simulink model "prensa_fluidtek"  (R2026b)
settings: Solver=ode15s  StopTime=P.t_fin  MaxStep=1e-4  RelTol=1e-5
InitFcn:
  | if ~exist('P','var'), P = params_prensa(); end
  | if ~exist('cmd','var'), cmd = [0 0; 1 0; 1 1; 4 1; 4 -1; 7 -1; 7 0; 100 0]; end
values from neighbouring files (symbols this model uses):
  P = struct()    [params_prensa.m]
settings Model: Creator=joela  LastModifiedBy=joela

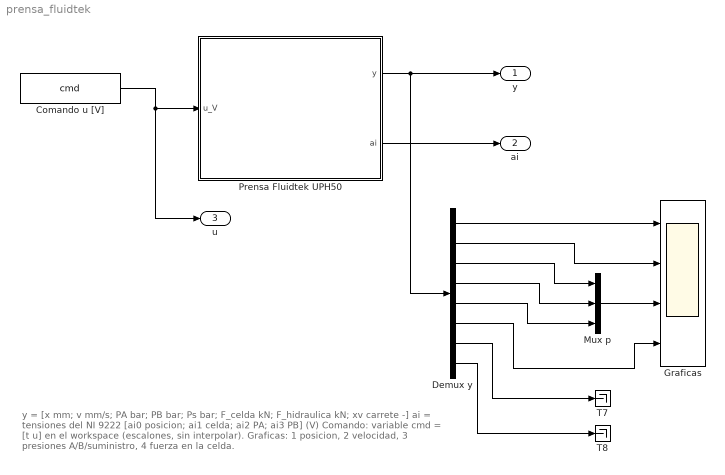
== system prensa_fluidtek ==
  note: y = [x mm; v mm/s; PA bar; PB bar; Ps bar; F_celda kN; F_hidraulica kN; xv carrete -]
      | ai = tensiones del NI 9222 [ai0 posicion; ai1 celda; ai2 PA; ai3 PB] (V)
      | Comando: variable cmd = [t u] en el workspace (escalones, sin interpolar).
      | Graficas: 1 posicion, 2 velocidad, 3 presiones A/B/suministro, 4 fuerza en la celda.
  Comando u [V] : FromWorkspace  VariableName=cmd  Interpolate=off  OutputAfterFinalValue=Holding final value
  Demux y : Demux  Outputs=8
  Graficas : Scope  NumInputPorts=4
  Mux p : Mux  Inputs=3
  Prensa Fluidtek UPH50 : Subsystem
  T7 : Terminator
  T8 : Terminator
  y : Outport
  ai : Outport  Port=2
  u : Outport  Port=3
  wires:
  Comando u [V]/1 -> Prensa Fluidtek UPH50/1(u_V), u/1
  Prensa Fluidtek UPH50/1(y) -> y/1, Demux y/1
  Prensa Fluidtek UPH50/2(ai) -> ai/1
  Demux y/1 -> Graficas/1
  Demux y/2 -> Graficas/2
  Demux y/3 -> Mux p/1
  Demux y/4 -> Mux p/2
  Demux y/5 -> Mux p/3
  Mux p/1 -> Graficas/3
  Demux y/6 -> Graficas/4
  Demux y/7 -> T7/1
  Demux y/8 -> T8/1

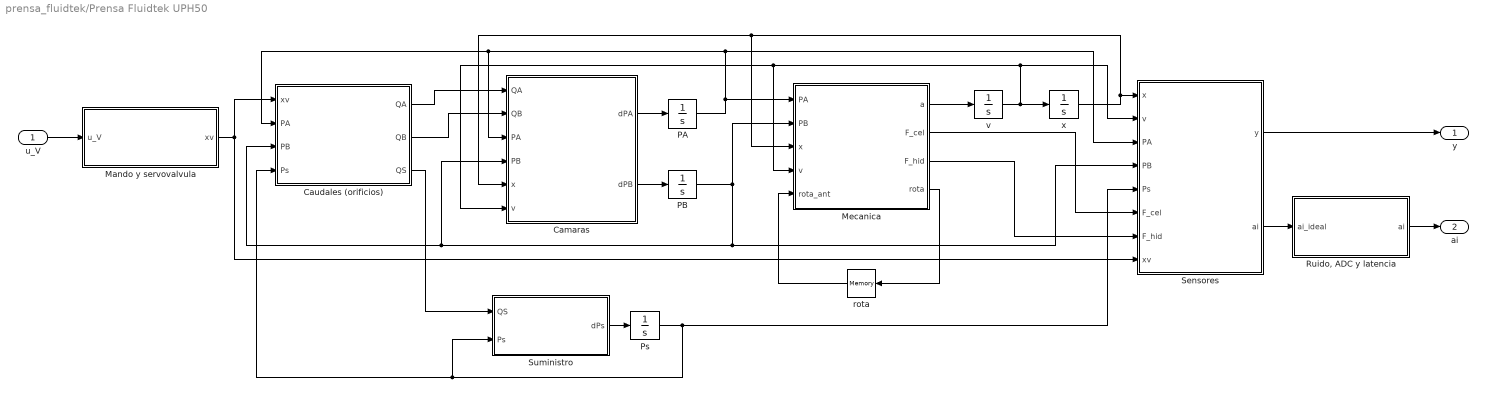
== system prensa_fluidtek/Prensa Fluidtek UPH50 ==
  u_V : Inport
  Camaras : MATLAB Function  TreatAsAtomicUnit=on
  Caudales (orificios) : MATLAB Function  TreatAsAtomicUnit=on
  Mando y servovalvula : Subsystem
  Mecanica : MATLAB Function  TreatAsAtomicUnit=on
  PA : Integrator  InitialCondition=P.PA_ini  LimitOutput=on  UpperSaturationLimit=500e5  LowerSaturationLimit=0
  PB : Integrator  InitialCondition=P.PB_ini  LimitOutput=on  UpperSaturationLimit=500e5  LowerSaturationLimit=0
  Ps : Integrator  InitialCondition=P.Ps_ini  LimitOutput=on  UpperSaturationLimit=400e5  LowerSaturationLimit=0
  "Ruido, ADC y latencia" : Subsystem
  Sensores : MATLAB Function  TreatAsAtomicUnit=on
  Suministro : MATLAB Function  TreatAsAtomicUnit=on
  rota : Memory
  v : Integrator  AbsoluteTolerance=1e-9
  x : Integrator  InitialCondition=P.x_ini  AbsoluteTolerance=1e-10
  y : Outport
  ai : Outport  Port=2
  wires:
  u_V/1 -> Mando y servovalvula/1(u_V)
  Mando y servovalvula/1(xv) -> Caudales (orificios)/1(xv), Sensores/8(xv)
  PA/1 -> Mecanica/1(PA), Camaras/3(PA), Caudales (orificios)/2(PA), Sensores/3(PA)
  PB/1 -> Sensores/4(PB), Camaras/4(PB), Caudales (orificios)/3(PB), Mecanica/2(PB)
  Ps/1 -> Caudales (orificios)/4(Ps), Suministro/2(Ps), Sensores/5(Ps)
  Caudales (orificios)/3(QS) -> Suministro/1(QS)
  Suministro/1(dPs) -> Ps/1
  Caudales (orificios)/1(QA) -> Camaras/1(QA)
  Caudales (orificios)/2(QB) -> Camaras/2(QB)
  x/1 -> Mecanica/3(x), Camaras/5(x), Sensores/1(x)
  v/1 -> x/1, Mecanica/4(v), Camaras/6(v), Sensores/2(v)
  Camaras/1(dPA) -> PA/1
  Camaras/2(dPB) -> PB/1
  rota/1 -> Mecanica/5(rota_ant)
  Mecanica/1(a) -> v/1
  Mecanica/4(rota) -> rota/1
  Mecanica/2(F_cel) -> Sensores/6(F_cel)
  Mecanica/3(F_hid) -> Sensores/7(F_hid)
  Sensores/1(y) -> y/1
  Sensores/2(ai) -> "Ruido, ADC y latencia"/1(ai_ideal)
  "Ruido, ADC y latencia"/1(ai) -> ai/1

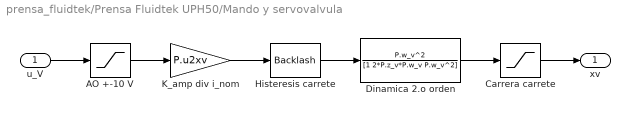
== system prensa_fluidtek/Prensa Fluidtek UPH50/Mando y servovalvula ==
  u_V : Inport
  AO +-10 V : Saturate  UpperLimit=P.u_max  LowerLimit=-P.u_max
  Carrera carrete : Saturate  UpperLimit=1  LowerLimit=-1
  Dinamica 2.o orden : TransferFcn  Numerator=P.w_v^2  Denominator=[1 2*P.z_v*P.w_v P.w_v^2]
  Histeresis carrete : Backlash  BacklashWidth=max(P.histeresis,1e-9)
  K_amp div i_nom : Gain  Gain=P.u2xv
  xv : Outport
  wires:
  u_V/1 -> AO +-10 V/1
  AO +-10 V/1 -> K_amp div i_nom/1
  K_amp div i_nom/1 -> Histeresis carrete/1
  Histeresis carrete/1 -> Dinamica 2.o orden/1
  Dinamica 2.o orden/1 -> Carrera carrete/1
  Carrera carrete/1 -> xv/1

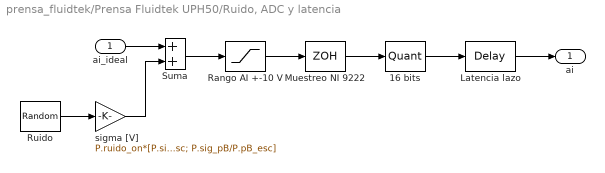
== system prensa_fluidtek/Prensa Fluidtek UPH50/Ruido, ADC y latencia ==
  ai_ideal : Inport
  16 bits : Quantizer  QuantizationInterval=20/2^16
  Latencia lazo : TransportDelay  DelayTime=P.latencia
  Muestreo NI 9222 : ZeroOrderHold  SampleTime=P.Ts_daq
  Rango AI +-10 V : Saturate  UpperLimit=10  LowerLimit=-10
  Ruido : RandomNumber  Seed=[11 12 13 14]  SampleTime=P.Ts_daq
  Suma : Sum
  sigma [V] : Gain  Gain=P.ruido_on*[P.sig_x/P.Kx_sens; P.sig_F/P.KF_sens; P.sig_pA/P.pA_esc; P.sig_pB/P.pB_esc]
  ai : Outport
  wires:
  ai_ideal/1 -> Suma/1
  Ruido/1 -> sigma [V]/1
  sigma [V]/1 -> Suma/2
  Suma/1 -> Rango AI +-10 V/1
  Rango AI +-10 V/1 -> Muestreo NI 9222/1
  Muestreo NI 9222/1 -> 16 bits/1
  16 bits/1 -> Latencia lazo/1
  Latencia lazo/1 -> ai/1

== matlab function prensa_fluidtek/Prensa Fluidtek UPH50/Suministro ==
  data: QS input; dPs output; Ps input; P parameter
function dPs = f_suministro(QS, Ps, P)
%#codegen
% Fuente de presion (Jelali 4.2.4): bomba de caudal constante Qp, limitadora
% tarada en Ps0, capacidad de la manguera P y del acumulador de vejiga.
if P.supply_dyn < 0.5
    dPs = 0;   % presion de suministro ideal y constante
    return
end
Qrv = P.K_rv*max(Ps - P.Ps0, 0);          % limitadora
C = P.V_s/E_lee(Ps, P);                    % aceite en manguera y manifold
if Ps > P.p_acc0                           % acumulador (gas politropico)
    Vg = P.V_acc*(P.p_acc0/Ps)^(1/P.n_acc);
    C = C + Vg/(P.n_acc*Ps);
end
dPs = (P.Qp - QS - Qrv)/C;
end

function E = E_lee(p, P)
% Modulo de compresibilidad efectivo de Lee (Jelali 3.21)
E = P.a1*P.E_max*log10(P.a2*max(p, 1e4)/P.p_max + P.a3);
end

== matlab function prensa_fluidtek/Prensa Fluidtek UPH50/Caudales (orificios) ==
  data: xv input; QA output; PA input; PB input; Ps input; QB output; QS output; P parameter
function [QA, QB, QS] = f_caudales(xv, PA, PB, Ps, P)
%#codegen
% Servovalvula de 4 vias, Jelali & Kroll (2003) ec. 4.5-4.6 (underlap).
% xv: posicion normalizada del carrete [-1,1]; presiones en Pa.
% QA = caudal que ENTRA en la camara A; QB = caudal que ENTRA en la camara B;
% QS = caudal que sale de la fuente de presion.
xe = xv + P.x0;                 % offset de null
a1 = max(P.xu + xe, 0);         % aristas P->A y B->T
a2 = max(P.xu - xe, 0);         % aristas P->B y A->T
QPA = P.Cv*a1*rq(Ps - PA, P.p_lam);
QAT = P.Cv*a2*rq(PA - P.PT, P.p_lam);
QPB = P.Cv*a2*rq(Ps - PB, P.p_lam);
QBT = P.Cv*a1*rq(PB - P.PT, P.p_lam);
QA = QPA - QAT;
QB = QPB - QBT;
QS = QPA + QPB;
end

function q = rq(dp, pl)
% raiz con signo: turbulenta si |dp| >> pl, laminar cerca de cero
q = dp/sqrt(abs(dp) + pl);
end

== matlab function prensa_fluidtek/Prensa Fluidtek UPH50/Camaras ==
  data: QA input; dPA output; QB input; PA input; PB input; x input; v input; dPB output; P parameter
function [dPA, dPB] = f_camaras(QA, QB, PA, PB, x, v, P)
%#codegen
% Dinamica de presion en las camaras, Jelali (2003) ec. 4.51-4.52.
% Volumenes variables con la carrera (4.46-4.47); x=0 vastago retraido.
VA = max(P.VA0 + P.A_A*x, 1e-6);
VB = max(P.VB0 + P.A_B*(P.L_fis - x), 1e-6);
QLi = P.C_Li*(PA - PB);                    % fuga interna laminar (4.55)
dPA = E_lee(PA, P)/VA*(QA - P.A_A*v - QLi);
dPB = E_lee(PB, P)/VB*(QB + P.A_B*v + QLi);
end

function E = E_lee(p, P)
% Modulo de compresibilidad efectivo de Lee (Jelali 3.21)
E = P.a1*P.E_max*log10(P.a2*max(p, 1e4)/P.p_max + P.a3);
end

== matlab function prensa_fluidtek/Prensa Fluidtek UPH50/Mecanica ==
  data: PA input; a output; PB input; x input; v input; rota_ant input; F_cel output; F_hid output; rota output; P parameter
function [a, F_cel, F_hid, rota] = f_mecanica(PA, PB, x, v, rota_ant, P)
%#codegen
% Ecuacion de movimiento, Jelali (2003) ec. 4.56, friccion de Stribeck 4.60.
% Montaje vertical: el peso W actua en +x (vastago saliendo hacia abajo).
F_hid = PA*P.A_A - PB*P.A_B;               % fuerza hidraulica (cilindro asimetrico)
Ff = P.sigma*v + tanh(v/P.v_eps)*(P.F_c + P.F_s*exp(-abs(v)/P.c_s));
% topes mecanicos elasticos (en vez del integrador con reset de Jelali 4.6.2)
F_tope = 0;
if x < 0
    F_tope = -P.k_stop*x - P.c_stop*min(v, 0);
elseif x > P.L_fis
    F_tope = -P.k_stop*(x - P.L_fis) - P.c_stop*max(v, 0);
end
% probeta: contacto elastico unilateral; al romper pierde la rigidez para siempre
rota = rota_ant;
F_cel = 0;
if P.k_p > 0 && rota_ant < 0.5 && x > P.x_c
    F_cel = P.k_p*(x - P.x_c);
    if F_cel >= P.F_rot
        rota = 1;
        F_cel = 0;
    end
end
a = (F_hid + P.W - Ff - F_cel + F_tope)/P.m;
end

== matlab function prensa_fluidtek/Prensa Fluidtek UPH50/Sensores ==
  data: x input; y output; v input; PA input; PB input; Ps input; F_cel input; F_hid input; xv input; ai output; P parameter
function [y, ai] = f_sensores(x, v, PA, PB, Ps, F_cel, F_hid, xv, P)
%#codegen
% Salidas en unidades de ingenieria y tensiones ideales de los canales AI.
y = [x*1e3; v*1e3; PA/1e5; PB/1e5; Ps/1e5; F_cel/1e3; F_hid/1e3; xv];
ai = [x*1e3/P.Kx_sens;                     % ai0 posicion (15 mm/V)
      F_cel/1e3/P.KF_sens;                  % ai1 celda (20 kN/V)
      P.pA_off + PA/1e5/P.pA_esc;           % ai2 presion A (calibrada)
      P.pB_off + PB/1e5/P.pB_esc];          % ai3 presion B (calibrada)
end
